simulink model "QEI_ADC3"  (Simulink 6.6)
settings: Solver=FixedStepDiscrete  StartTime=0.0  StopTime=10.0  FixedStep=0.001  RelTol=1e-3
undefined symbols (not defined in the file or in its folder): QEIInit
libraries: dsPICdrivers x9, simulink x2
settings Model: Creator=123  LastModifiedBy=123  ProdHWDeviceType=16-bit Generic
settings OptimizationCC: OptimizeModelRefInitCode=on  LifeSpan=1
settings HardwareCC: ProdBitPerInt=16  ProdEndianess=LittleEndian  ProdWordSize=16  ProdHWDeviceType=16-bit Generic  TargetHWDeviceType=32-bit Generic
settings RTWCC: SystemTargetFile=dspic.tlc  TemplateMakefile=dspic_pic30_gcc.tmf  PostCodeGenCommand=dsPIC_Compile()  Description=Embedded Target for Microchip dsPIC (real-time)  ProcessScript=dspic_make_rtw_hook  CustomSource=myQEI.c
settings CodeAppCC: IgnoreCustomStorageClasses=off
settings STFCustomTargetCC: TargetFcnLib=ansi_tfl_tmw.mat  GenFloatMathFcnCalls=ANSI_C  ModelReferenceCompliant=off  IncludeMdlTerminateFcn=off  CombineOutputUpdateFcns=on  SuppressErrorStatus=on  ERTCustomFileBanners=on  SupportContinuousTime=off  SupportNonInlinedSFcns=off  SystemTargetFile=dspic.tlc
settings ERTTargetCC: TargetFcnLib=ansi_tfl_tmw.mat  GenFloatMathFcnCalls=ANSI_C  ModelReferenceCompliant=off  IncludeMdlTerminateFcn=off  SuppressErrorStatus=on  ModelStepFunctionPrototypeControlCompliant=off  InlinedParameterPlacement=NonHierarchical  ERTSrcFileBannerTemplate=dsPIC_code_template.cgt  ERTHdrFileBannerTemplate=dsPIC_code_template.cgt  ERTDataSrcFileTemplate=dsPIC_code_template.cgt  ERTDataHdrFileTemplate=dsPIC_code_template.cgt  ERTCustomFileTemplate=dsPIC_main.tlc
settings CustomProperty: DataType=string  Value=C:\PROGRA~2\MATLAB\R2007a\rtw\bin\win32\gmake

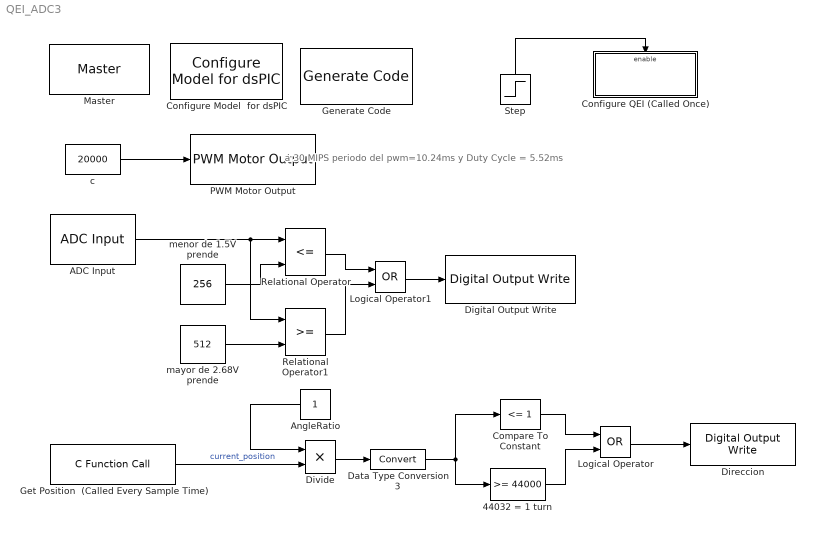
== system QEI_ADC3 ==
  note: a 30 MIPS periodo del pwm=10.24ms
      | y Duty Cycle = 5.52ms
  "44032 = 1 turn " : simulink/Logic and Bit Operations/Compare To Constant  SystemSampleTime=-1  relop=>=  const=44000  LogicOutDataTypeMode=boolean  ZeroCross=off
  ADC Input : dsPICdrivers/Peripheral I//O/ADC Input  Tag=dsPIC_ADC  Priority=5  ADC_TYPE=10 bits  ADC_MODE=Continuous sampling & get last channel value  NbrSampleStep=1  VoltRefpopup="AVdd  -  AVss"  OutFormatBitspopup=0000 00dd dddd dddd : Integer  InterruptPriority=1  ANCHANNELS=[0]  MaxName=ANmax = 1024  Rin=1e2  ADCS=9  SAMC=1  Temperature=25  DMAChannel=0  SampleTime=.001  Status="OK  |  Tsmp=1.667e-007 |  T/Channel=2.167e-006 |  Tall=2.167e-006"
  AngleRatio : Constant  Orientation=left  SampleTime=.001
  Compare To Constant : simulink/Logic and Bit Operations/Compare To Constant  SystemSampleTime=-1  relop=<=  const=1  LogicOutDataTypeMode=boolean  ZeroCross=off
  Configure Model  for dsPIC : dsPICdrivers/Simulink Configuration/Configure Model  for dsPIC
  Configure QEI (Called Once) : Subsystem  TreatAsAtomicUnit=on
  Data Type Conversion3 : DataTypeConversion  OutDataTypeMode=int32  SampleTime=.001
  Digital Output Write : dsPICdrivers/Digital I//O/Digital Output Write  Tag=dsPIC_Digital_Output  Priority=5  PORT=D  Pin=[0]  Simultaneous=off  OrderingInOutPopup=None
  Direccion : dsPICdrivers/Digital I//O/Digital Output Write  Tag=dsPIC_Digital_Output  Priority=5  PORT=D  Pin=[1]  Simultaneous=off  OrderingInOutPopup=None
  Divide : Product  Inputs=**  OutScaling=2^-10  SampleTime=.001
  Generate Code : dsPICdrivers/Simulink Configuration/Generate Code
  Get Position  (Called Every Sample Time) : dsPICdrivers/OTHERS/C Function Call  Tag=dsPIC_dsPIC_CFunctionCall  fctName='GetQEI'  INPUT_SIZE=1  INPUT1=--  INPUT2=--  INPUT3=--  OUTPUT_SIZE=1  OUTPUT1=int32  SampleTime=.001  InputType=[ ]  OutputType=[ 5 ]  FctDeclaration=extern int32_T GetQEI();  FctCall=%y1 = GetQEI();  OrderingInOutPopup=None
  Logical Operator : Logic  Operator=OR  AllPortsSameDT=off  OutDataTypeMode=Boolean  SampleTime=.001
  Logical Operator1 : Logic  Operator=OR  AllPortsSameDT=off  OutDataTypeMode=Boolean  SampleTime=.001
  Master : dsPICdrivers/Master  Tag=dsPIC_MASTER  Priority=1  TimeStepType=Timer1  picType=30f4012  fcy=30e6  Quartz_33f=5e6  PLLActive_33f=off  fcyDesired_33f=0  tmr1="[1  29999  0]"  tmr1Info="Time Step : 0.001  ;   Error : 0%  PR1=29999"  tmr2345="[0  0  0  0]"  tmr2345cfg=[-1 -1 -1 -1]  IOautoConf=on  typePort="[ 0   0   0   0   0   0   0   0   0   0   0   0   0   0   0   0   8   0   0   0   0   0   0   0   0   0   0   0   0   0   0   0   0   0   0   0   0   0   0   0   0   0   0   0   0   0   0   0  10  10   0   0   0   0   0   0   0   0   0   0   0   0   0   0  11   0   0   0   0   0   0   0   0   0   0   0   0   0   0   0   0   0   0   0   0   0   0   0   0   0   0   0   0   0   0   0   0   0   0   0   0   0   0   0   0   0   0   0   0   0   0   0 ]"  TRIS="[ 65535  65535  65535  65532  65535  65535  65535 ]"  ADPCFG=0  MasterBusyPort=None  MasterOverloadPort=None  FOSC=FRC_PLL16  ClockSwitchMonitor=Both disabled  TempProtection_33f=TEMP_ON  FPBOR=PBOR_OFF  PWRT=PWRT_OFF  MCLR=MCLR_DIS  PowerSave=off  OverrideFcy=off  NewFcy=1e6
  PWM Motor Output : dsPICdrivers/Peripheral I//O/PWM Motor Output  Tag=dsPIC_PWM_Motor  Priority=5  InputEnableChk=off  InputPeriodeChk=off  Channel=[1 ]  TPeriode=.01  PrescalerValue=16  PeriodeInteger=18750  MaxName='PWM'  Centered=off  HChannelON=off  Info="Nbr Bits : 15.1946  ||  PWM = 37500  ||  Prescaler = 16"  Delay=0  IntPriority=5  nbrPwmChannelPIC=3  Status=OK
  Relational Operator : RelationalOperator  Operator=<=  LogicOutDataTypeMode=Boolean  SampleTime=.001
  Relational Operator1 : RelationalOperator  LogicOutDataTypeMode=Boolean  SampleTime=.001
  Step : Step  Orientation=up  Time=0.002  Before=1  After=0  SampleTime=0.001
  c : Constant  Value=20000  OutDataTypeMode=uint16  SampleTime=.001
  mayor de 2.68V prende : Constant  Value=512  OutDataTypeMode=uint16  SampleTime=.001
  menor de 1.5V prende : Constant  Value=256  OutDataTypeMode=uint16  SampleTime=.001
  wires:
  c/1 -> PWM Motor Output/1
  menor de 1.5V prende/1 -> Relational Operator/2
  ADC Input/1 -> Relational Operator/1, Relational Operator1/1
  mayor de 2.68V prende/1 -> Relational Operator1/2
  Relational Operator/1 -> Logical Operator1/1
  Relational Operator1/1 -> Logical Operator1/2
  Logical Operator1/1 -> Digital Output Write/1
  AngleRatio/1 -> Divide/1
  Divide/1 -> Data Type Conversion3/1
  Get Position  (Called Every Sample Time)/1 -> Divide/2  "current_position"
  Compare To Constant/1 -> Logical Operator/1
  "44032 = 1 turn "/1 -> Logical Operator/2
  Logical Operator/1 -> Direccion/1
  Data Type Conversion3/1 -> Compare To Constant/1, "44032 = 1 turn "/1
  Step/1 -> Configure QEI (Called Once)/Enable

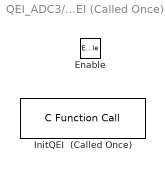
== system QEI_ADC3/Configure QEI (Called Once) ==
  Enable : EnablePort
  InitQEI  (Called Once) : dsPICdrivers/OTHERS/C Function Call  Tag=dsPIC_dsPIC_CFunctionCall  fctName='QEIInit'  INPUT_SIZE=1  INPUT1=--  INPUT2=--  INPUT3=--  OUTPUT_SIZE=1  OUTPUT1=--  SampleTime=inf  InputType=[ ]  OutputType=[ ]  FctDeclaration=extern void QEIInit();  FctCall=QEIInit();  OrderingInOutPopup=None
